simulink model "F2026_ECE597_01_Closed_Loop_Step_Response_LQR"  (R2025a)
settings: Solver=VariableStepAuto  StartTime=0.0  StopTime=60.0  RelTol=1e-3
values from neighbouring files (symbols this model uses):
  A = [[-0.59 0.92 0.61 -9.82]; [-0.23 -6.31 4.42 0.19]; [ 0.78 -5.59 -5.92 0]; [0 0 1 0]]    [F2026_ECE597_01_Closed_Loop_Step_Response_LQR_Driver.m]
  B = B_w_wind(:,1:2)    [F2026_ECE597_01_Closed_Loop_Step_Response_LQR_Driver.m]
  C = [[1 0 0 0]; [0 0 0 1]]    [F2026_ECE597_01_Closed_Loop_Step_Response_LQR_Driver.m]
  elevator_max = deg2rad(20) - elevator_init    [F2026_ECE597_01_Closed_Loop_Step_Response_LQR_Driver.m]
  elevator_min = -deg2rad(20) - elevator_init    [F2026_ECE597_01_Closed_Loop_Step_Response_LQR_Driver.m]
  forward_airspeed_disturbance_gain = 0.5    [F2026_ECE597_01_Closed_Loop_Step_Response_LQR_Driver.m]
  K = lqr(G, Q, R)    [F2026_ECE597_01_Closed_Loop_Step_Response_LQR_Driver.m]
  pitch_disturbance_gain = 10 * (pi/180)    (= 0.174532925199)    [F2026_ECE597_01_Closed_Loop_Step_Response_LQR_Driver.m]
  pitch_rate_disturbance_gain = 10.0    (= 10)    [F2026_ECE597_01_Closed_Loop_Step_Response_LQR_Driver.m]
  throttle_max = 1.0 - throttle_init    (= 0.56)    [F2026_ECE597_01_Closed_Loop_Step_Response_LQR_Driver.m]
  throttle_min = 0.0 - throttle_init    (= -0.44)    [F2026_ECE597_01_Closed_Loop_Step_Response_LQR_Driver.m]
  vertical_airspeed_disturbance_gain = 3.0    (= 3)    [F2026_ECE597_01_Closed_Loop_Step_Response_LQR_Driver.m]
libraries: dspsrcs4 x1
settings Model: Creator=gresham2  LastModifiedBy=gresham2

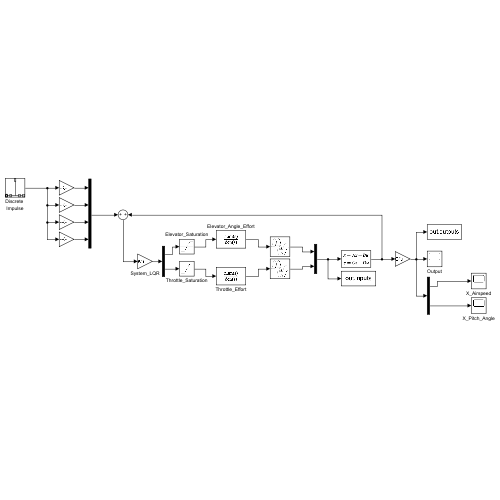
[thumbnail: Simulink's stored preview of the top-level diagram]
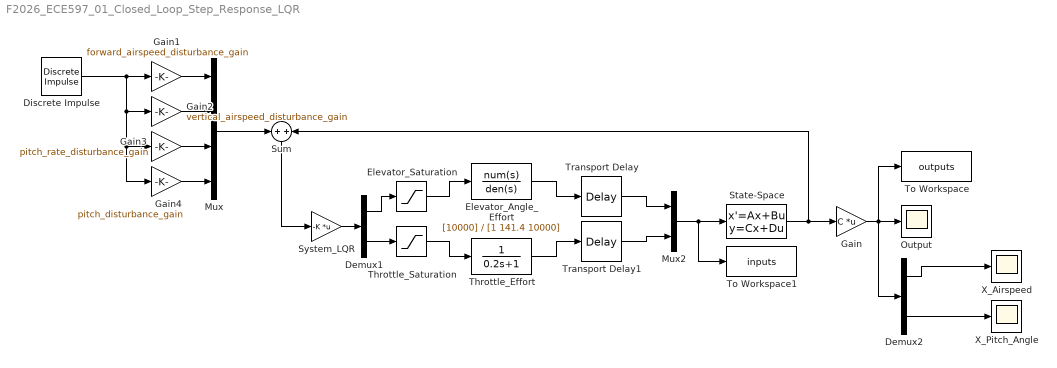
== system F2026_ECE597_01_Closed_Loop_Step_Response_LQR ==
  Demux1 : Demux  Outputs=2
  Demux2 : Demux  Outputs=2
  Discrete Impulse : dspsrcs4/Discrete  Impulse  Delay=0  SampleTime=1  FrameSample=1  OutputFrames=off  dataType=double  isSigned=on  wordLen=16  udDataType=sfix(16)  fracBitsMode=Best precision  numFracBits=15  OutDataTypeStr=double  LastOutDataTypeStr=double
  Elevator_Angle_Effort : TransferFcn  Numerator=[10000]  Denominator=[1 141.4 10000]
  Elevator_Saturation : Saturate  UpperLimit=elevator_max  LowerLimit=elevator_min
  Gain : Gain  Gain=C  Multiplication=Matrix(K*u)
  Gain1 : Gain  Gain=forward_airspeed_disturbance_gain
  Gain2 : Gain  Gain=vertical_airspeed_disturbance_gain
  Gain3 : Gain  Gain=pitch_rate_disturbance_gain
  Gain4 : Gain  Gain=pitch_disturbance_gain
  Mux : Mux
  Mux2 : Mux  Inputs=2
  Output : Scope
      settings: ActiveDisplayYMinimum=-1  ActiveDisplayYMaximum=1
  State-Space : StateSpace  A=A  B=B  C=eye(4)  D=zeros(4, 2)  InitialCondition=0
  Sum : Sum  Inputs=+|+
  System_LQR : Gain  Gain=-K  Multiplication=Matrix(K*u)
  Throttle_Effort : TransferFcn  Denominator=[0.2 1]
  Throttle_Saturation : Saturate  UpperLimit=throttle_max  LowerLimit=throttle_min
  To Workspace : ToWorkspace  VariableName=outputs  SaveFormat=Timeseries  SampleTime=-1
  To Workspace1 : ToWorkspace  VariableName=inputs  SaveFormat=Timeseries  SampleTime=-1
  Transport Delay : TransportDelay  DelayTime=0.07
  Transport Delay1 : TransportDelay  DelayTime=0.05
  X_Airspeed : Scope
      settings: ActiveDisplayYMinimum=-1  ActiveDisplayYMaximum=1  DataLoggingVariableName=ScopeData4
  X_Pitch_Angle : Scope
      settings: ActiveDisplayYMinimum=-1  ActiveDisplayYMaximum=1  DataLoggingVariableName=ScopeData3
  wires:
  Demux2/1 -> X_Airspeed/1
  Demux2/2 -> X_Pitch_Angle/1
  Demux1/2 -> Throttle_Saturation/1
  Demux1/1 -> Elevator_Saturation/1
  Mux2/1 -> To Workspace1/1, State-Space/1
  Elevator_Angle_Effort/1 -> Transport Delay/1
  Throttle_Effort/1 -> Transport Delay1/1
  Elevator_Saturation/1 -> Elevator_Angle_Effort/1
  Throttle_Saturation/1 -> Throttle_Effort/1
  Transport Delay/1 -> Mux2/1
  Transport Delay1/1 -> Mux2/2
  State-Space/1 -> Sum/2, Gain/1
  Gain/1 -> Demux2/1, To Workspace/1, Output/1
  Gain1/1 -> Mux/1
  Discrete Impulse/1 -> Gain4/1, Gain3/1, Gain2/1, Gain1/1
  Gain2/1 -> Mux/2
  Gain4/1 -> Mux/4
  Gain3/1 -> Mux/3
  System_LQR/1 -> Demux1/1
  Sum/1 -> System_LQR/1
  Mux/1 -> Sum/1
